simulink model "DCMotor_M1_OpenLoop"  (R2026b)
settings: Solver=FixedStepDiscrete  StopTime=OL_StopTime  FixedStep=Ts
PreLoadFcn:
  | DCMotorParams;
InitFcn:
  | DCMotorParams;
values from neighbouring files (symbols this model uses):
  OL_Duty = [0 100   0 -100   0   0]    [DCMotorParams.m]
  OL_Scale = 1    [DCMotorParams.m]
  OL_Time = [0   2   6   9   13  16]    [DCMotorParams.m]
  Ts = 0.01    [DCMotorParams.m]
settings Model: SILPILModeSetting=veronly  SimulationMode=external  Creator=bence  LastModifiedBy=bence
settings OptimizationCC: DifferentSizesBufferReuse=on  EfficientTunableParamExpr=on  EnhancedBackFolding=on  MaxStackSize=64  OptimizationCustomize=off  OptimizeBlockOrder=speed  PassReuseOutputArgsAs=Individual arguments  RemoveInternalMemoryZeroInit=on  RemoveRootLevelIOMemoryZeroInit=on
settings DebuggingCC: ParameterTunabilityLossMsg=error
settings HardwareCC: ProdHWDeviceType=Atmel->AVR  ProdLargestAtomicFloat=None
settings SFSimCC: MATLABDynamicMemAlloc=off
settings RTWCC: BuildConfiguration=Faster Runs  Description=Embedded Coder  HardwareBoard=Arduino Uno  SystemTargetFile=ert.tlc  TLCOptions=-aInlineSetEventsForThisBaseRateFcn=TLC_FALSE -aSuppressMultiTaskScheduler=TLC_FALSE -aRateBasedStepFcn=1  TemplateMakefile=ert_default_tmf  Toolchain=Arduino AVR
settings CodeAppCC: ForceParamTrailComments=on  IgnoreCustomStorageClasses=off  InsertBlockDesc=on  OperatorAnnotations=on  SFDataObjDesc=on  SimulinkDataObjDesc=on
settings ERTTargetCC: CombineSignalStateStructs=on  ExtMode=on  ExtModeAutomaticAllocSize=off  ExtModeIntrfLevel=Level2 - Open  ExtModeMexFile=ext_xcp  ExtModeStaticAlloc=on  SupportContinuousTime=on  SupportVariableSizeSignals=on

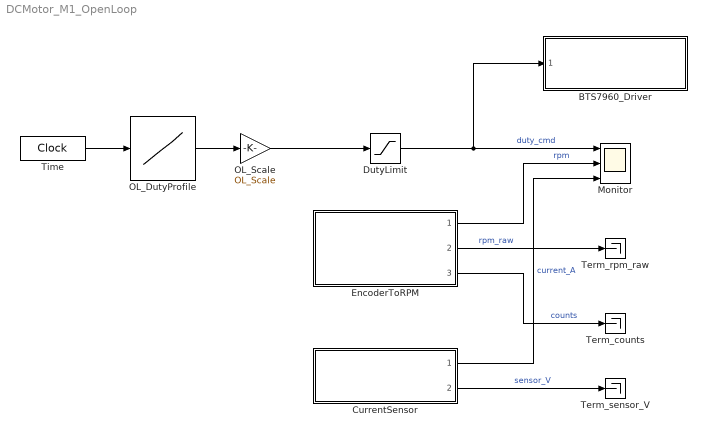
== system DCMotor_M1_OpenLoop ==
  BTS7960_Driver : Subsystem  ReferencedSubsystem=DC7960MDriver
  CurrentSensor : Subsystem  ReferencedSubsystem=CurrentSensor
  DutyLimit : Saturate  UpperLimit=100  LowerLimit=-100
  EncoderToRPM : Subsystem  ReferencedSubsystem=EncoderToRPM
  Monitor : Scope  NumInputPorts=3
      settings: ActiveDisplayYMinimum=-2774.75927734375  ActiveDisplayYMaximum=2739.22509765625
  OL_DutyProfile : Lookup_n-D  NumberOfTableDimensions=1  BreakpointsForDimension1=OL_Time  Table=OL_Duty  InterpMethod=Flat  ExtrapMethod=Clip  InternalRulePriority=Speed  RndMeth=Simplest
  OL_Scale : Gain  Gain=OL_Scale
  Term_counts : Terminator
  Term_rpm_raw : Terminator
  Term_sensor_V : Terminator
  Time : DigitalClock  SampleTime=Ts
  wires:
  CurrentSensor/2 -> Term_sensor_V/1  "sensor_V"
  CurrentSensor/1 -> Monitor/3  "current_A"
  EncoderToRPM/3 -> Term_counts/1  "counts"
  EncoderToRPM/2 -> Term_rpm_raw/1  "rpm_raw"
  EncoderToRPM/1 -> Monitor/2  "rpm"
  DutyLimit/1 -> BTS7960_Driver/1, Monitor/1  "duty_cmd"
  OL_Scale/1 -> DutyLimit/1
  OL_DutyProfile/1 -> OL_Scale/1
  Time/1 -> OL_DutyProfile/1
